simulink model "ADS_v1"  (R2026a)
settings: Solver=FixedStepDiscrete  StopTime=3600  FixedStep=ADS_P.dt
PostLoadFcn:
  | run(fullfile(fileparts(get_param('ADS_v1', 'FileName')), 'ads_setup.m'));
InitFcn:
  | run(fullfile(fileparts(get_param('ADS_v1', 'FileName')), 'ads_setup.m'));
values from neighbouring files (symbols this model uses):
  ADS_P = ads_params()    [ads_setup.m]
settings Model: Creator=Administrator  LastModifiedBy=Administrator

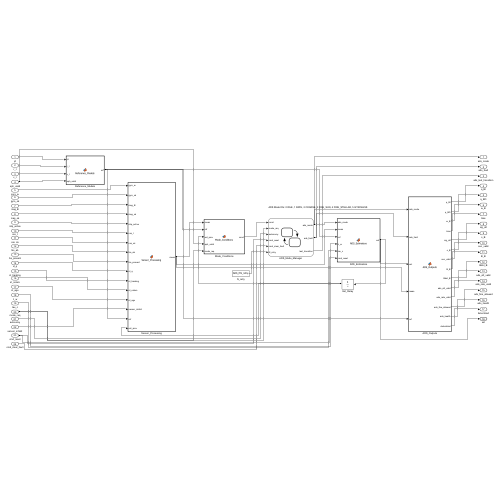
[thumbnail: Simulink's stored preview of the top-level diagram]
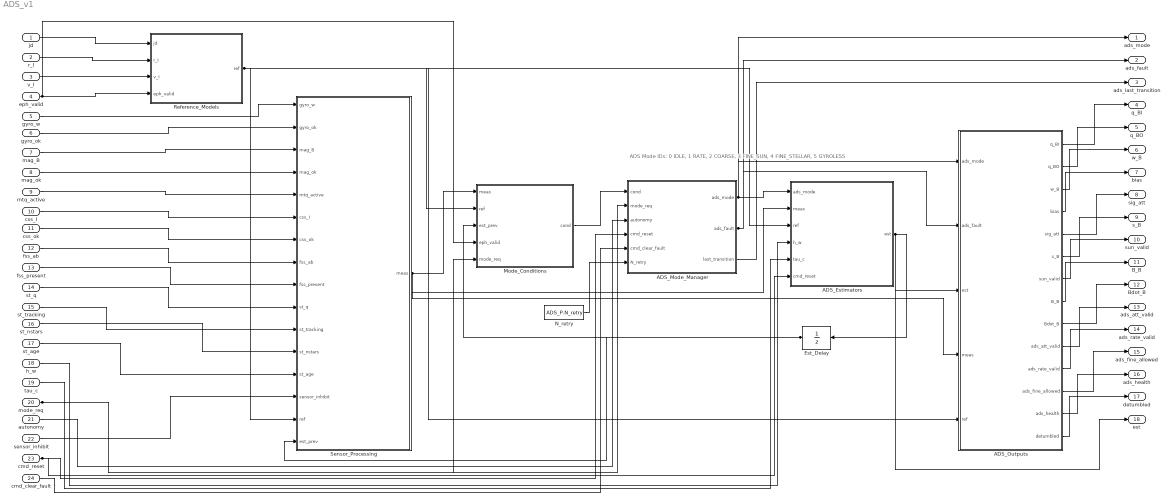
== system ADS_v1 ==
  note: ADS Mode IDs: 0 IDLE, 1 RATE, 2 COARSE, 3 FINE_SUN, 4 FINE_STELLAR, 5 GYROLESS
  jd : Inport  OutDataTypeStr=double  PortDimensions=1
  r_I : Inport  Port=2  OutDataTypeStr=double  PortDimensions=3
  v_I : Inport  Port=3  OutDataTypeStr=double  PortDimensions=3
  eph_valid : Inport  Port=4  OutDataTypeStr=boolean  PortDimensions=1
  gyro_w : Inport  Port=5  OutDataTypeStr=double  PortDimensions=3
  gyro_ok : Inport  Port=6  OutDataTypeStr=boolean  PortDimensions=1
  mag_B : Inport  Port=7  OutDataTypeStr=double  PortDimensions=3
  mag_ok : Inport  Port=8  OutDataTypeStr=boolean  PortDimensions=1
  mtq_active : Inport  Port=9  OutDataTypeStr=boolean  PortDimensions=1
  css_I : Inport  Port=10  OutDataTypeStr=double  PortDimensions=6
  css_ok : Inport  Port=11  OutDataTypeStr=boolean  PortDimensions=1
  fss_ab : Inport  Port=12  OutDataTypeStr=double  PortDimensions=4
  fss_present : Inport  Port=13  OutDataTypeStr=boolean  PortDimensions=2
  st_q : Inport  Port=14  OutDataTypeStr=double  PortDimensions=4
  st_tracking : Inport  Port=15  OutDataTypeStr=boolean  PortDimensions=1
  st_nstars : Inport  Port=16  OutDataTypeStr=double  PortDimensions=1
  st_age : Inport  Port=17  OutDataTypeStr=double  PortDimensions=1
  h_w : Inport  Port=18  OutDataTypeStr=double  PortDimensions=3
  tau_c : Inport  Port=19  OutDataTypeStr=double  PortDimensions=3
  mode_req : Inport  Port=20  OutDataTypeStr=uint8  PortDimensions=1
  autonomy : Inport  Port=21  OutDataTypeStr=boolean  PortDimensions=1
  sensor_inhibit : Inport  Port=22  OutDataTypeStr=uint8  PortDimensions=1
  cmd_reset : Inport  Port=23  OutDataTypeStr=boolean  PortDimensions=1
  cmd_clear_fault : Inport  Port=24  OutDataTypeStr=boolean  PortDimensions=1
  ADS_Estimators : MATLAB Function  TreatAsAtomicUnit=on
  ADS_Mode_Manager : Stateflow chart  TreatAsAtomicUnit=on
  ADS_Outputs : MATLAB Function  TreatAsAtomicUnit=on
  Est_Delay : UnitDelay  SampleTime=-1
  Mode_Conditions : MATLAB Function  TreatAsAtomicUnit=on
  N_retry : Constant  Value=ADS_P.N_retry  OutDataTypeStr=double  SampleTime=-1
  Reference_Models : MATLAB Function  TreatAsAtomicUnit=on
  Sensor_Processing : MATLAB Function  TreatAsAtomicUnit=on
  ads_mode : Outport
  ads_fault : Outport  Port=2
  ads_last_transition : Outport  Port=3
  q_BI : Outport  Port=4
  q_BO : Outport  Port=5
  w_B : Outport  Port=6
  bias : Outport  Port=7
  sig_att : Outport  Port=8
  s_B : Outport  Port=9
  sun_valid : Outport  Port=10
  B_B : Outport  Port=11
  Bdot_B : Outport  Port=12
  ads_att_valid : Outport  Port=13
  ads_rate_valid : Outport  Port=14
  ads_fine_allowed : Outport  Port=15
  ads_health : Outport  Port=16
  detumbled : Outport  Port=17
  est : Outport  Port=18  OutDataTypeStr=Bus: ADS_EstBus
  wires:
  jd/1 -> Reference_Models/1(jd)
  r_I/1 -> Reference_Models/2(r_I)
  v_I/1 -> Reference_Models/3(v_I)
  eph_valid/1 -> Reference_Models/4(eph_valid), Mode_Conditions/4(eph_valid)
  gyro_w/1 -> Sensor_Processing/1(gyro_w)
  gyro_ok/1 -> Sensor_Processing/2(gyro_ok)
  mag_B/1 -> Sensor_Processing/3(mag_B)
  mag_ok/1 -> Sensor_Processing/4(mag_ok)
  mtq_active/1 -> Sensor_Processing/5(mtq_active)
  css_I/1 -> Sensor_Processing/6(css_I)
  css_ok/1 -> Sensor_Processing/7(css_ok)
  fss_ab/1 -> Sensor_Processing/8(fss_ab)
  fss_present/1 -> Sensor_Processing/9(fss_present)
  st_q/1 -> Sensor_Processing/10(st_q)
  st_tracking/1 -> Sensor_Processing/11(st_tracking)
  st_nstars/1 -> Sensor_Processing/12(st_nstars)
  st_age/1 -> Sensor_Processing/13(st_age)
  sensor_inhibit/1 -> Sensor_Processing/14(sensor_inhibit)
  Reference_Models/1(ref) -> Sensor_Processing/15(ref), Mode_Conditions/2(ref), ADS_Estimators/3(ref), ADS_Outputs/5(ref)
  Est_Delay/1 -> Sensor_Processing/16(est_prev), Mode_Conditions/3(est_prev)
  Sensor_Processing/1(meas) -> Mode_Conditions/1(meas), ADS_Estimators/2(meas), ADS_Outputs/4(meas)
  mode_req/1 -> Mode_Conditions/5(mode_req), ADS_Mode_Manager/2(mode_req)
  Mode_Conditions/1(cond) -> ADS_Mode_Manager/1(cond)
  autonomy/1 -> ADS_Mode_Manager/3(autonomy)
  cmd_reset/1 -> ADS_Mode_Manager/4(cmd_reset), ADS_Estimators/6(cmd_reset)
  cmd_clear_fault/1 -> ADS_Mode_Manager/5(cmd_clear_fault)
  N_retry/1 -> ADS_Mode_Manager/6(N_retry)
  ADS_Mode_Manager/1(ads_mode) -> ADS_Estimators/1(ads_mode), ADS_Outputs/1(ads_mode), ads_mode/1
  h_w/1 -> ADS_Estimators/4(h_w)
  tau_c/1 -> ADS_Estimators/5(tau_c)
  ADS_Estimators/1(est) -> Est_Delay/1, ADS_Outputs/3(est), est/1
  ADS_Mode_Manager/2(ads_fault) -> ADS_Outputs/2(ads_fault), ads_fault/1
  ADS_Mode_Manager/3(last_transition) -> ads_last_transition/1
  ADS_Outputs/1(q_BI) -> q_BI/1
  ADS_Outputs/2(q_BO) -> q_BO/1
  ADS_Outputs/3(w_B) -> w_B/1
  ADS_Outputs/4(bias) -> bias/1
  ADS_Outputs/5(sig_att) -> sig_att/1
  ADS_Outputs/6(s_B) -> s_B/1
  ADS_Outputs/7(sun_valid) -> sun_valid/1
  ADS_Outputs/8(B_B) -> B_B/1
  ADS_Outputs/9(Bdot_B) -> Bdot_B/1
  ADS_Outputs/10(ads_att_valid) -> ads_att_valid/1
  ADS_Outputs/11(ads_rate_valid) -> ads_rate_valid/1
  ADS_Outputs/12(ads_fine_allowed) -> ads_fine_allowed/1
  ADS_Outputs/13(ads_health) -> ads_health/1
  ADS_Outputs/14(detumbled) -> detumbled/1

== matlab function ADS_v1/Sensor_Processing ==
  data: gyro_w input; meas output Bus: ADS_MeasBus; gyro_ok input; mag_B input; mag_ok input; mtq_active input; css_I input; css_ok input; fss_ab input; fss_present input; st_q input; st_tracking input; st_nstars input; st_age input; sensor_inhibit input; ref input Bus: ADS_RefBus; est_prev input Bus: ADS_EstBus; ADS_P parameter
function meas = Sensor_Processing(gyro_w, gyro_ok, mag_B, mag_ok, mtq_active, css_I, css_ok, fss_ab, fss_present, st_q, st_tracking, st_nstars, st_age, sensor_inhibit, ref, est_prev, ADS_P)
% Calibration, frame transformation and validity checks (Sections 3, 12.1).
meas = ads_sensor_processing(gyro_w, gyro_ok, mag_B, mag_ok, mtq_active, css_I, css_ok, fss_ab, fss_present, st_q, st_tracking, st_nstars, st_age, sensor_inhibit, ref, est_prev, ADS_P);

== matlab function ADS_v1/Reference_Models ==
  data: jd input; ref output Bus: ADS_RefBus; r_I input; v_I input; eph_valid input; ADS_P parameter
function ref = Reference_Models(jd, r_I, v_I, eph_valid, ADS_P)
% Sun, eclipse, IGRF field and LVLH frame (Section 3.7).
ref = ads_reference_models(jd, r_I, v_I, eph_valid, ADS_P);

== matlab function ADS_v1/Mode_Conditions ==
  data: meas input Bus: ADS_MeasBus; cond output Bus: ADS_CondBus; ref input Bus: ADS_RefBus; est_prev input Bus: ADS_EstBus; eph_valid input; mode_req input; ADS_P parameter
function cond = Mode_Conditions(meas, ref, est_prev, eph_valid, mode_req, ADS_P)
% Persistence-filtered guard conditions for transitions T1-T15 (Section 4.3).
cond = ads_mode_conditions(meas, ref, est_prev, eph_valid, mode_req, ADS_P);

== stateflow chart ADS_v1/ADS_Mode_Manager ==
  settings: enableNonTerminalStates=1
  state ADS_ACTIVE
    state ADS_FINE_STELLAR
      entry: ads_mode = uint8(4);
      during: bookkeeping();
    state ADS_FINE_SUN
      entry: ads_mode = uint8(3);
      during: bookkeeping();
    state ADS_COARSE
      entry: ads_mode = uint8(2);
      during: bookkeeping();
    state ADS_GYROLESS
      entry: ads_mode = uint8(5);
      during: bookkeeping();
    state ADS_RATE
      entry: ads_mode = uint8(1);
      during: bookkeeping();
    ADS_FINE_STELLAR -> ADS_GYROLESS [order 1] : [T11()]{fault_fb(11)}
    ADS_COARSE -> ADS_FINE_STELLAR [order 5] : [T10()]{mark(10)}
    (junction 73) -> ADS_FINE_STELLAR [order 1] : [T14_FST()]{mark(14)}
    ADS_RATE -> ADS_FINE_STELLAR [order 1] : [T10()]{mark(10)}
    ADS_FINE_STELLAR -> ADS_COARSE [order 2] : [T9f()]{fault_fb(9)}
    ADS_FINE_STELLAR -> ADS_COARSE [order 4] : [T9g()]{mark(9)}
    ADS_FINE_SUN -> ADS_FINE_STELLAR [order 5] : [T7()]{mark(7)}
    ADS_FINE_STELLAR -> (junction 72) [order 5] : [cond.req_rank < 5]{mark(16)}
    ADS_FINE_STELLAR -> ADS_FINE_SUN [order 3] : [T8()]{mark(8)}
    (junction 73) -> ADS_FINE_SUN [order 2] : [T14_FSUN()]{mark(14)}
    (junction 73) -> ADS_COARSE [order 3] : [T14_CRS()]{mark(14)}
    ADS_GYROLESS -> (junction 73) [order 4] : [T14()]
    ADS_FINE_SUN -> ADS_GYROLESS [order 1] : [T11()]{fault_fb(11)}
    (default) -> ADS_RATE
    ADS_COARSE -> ADS_FINE_SUN [order 6] : [T5()]{mark(5)}
    ADS_FINE_SUN -> ADS_COARSE [order 3] : [T6g()]{mark(6)}
    ADS_FINE_SUN -> (junction 72) [order 4] : [cond.req_rank < 4]{mark(16)}
    ADS_FINE_SUN -> ADS_COARSE [order 2] : [T6f()]{fault_fb(6)}
    (junction 72) -> ADS_FINE_SUN [order 4] : [mode_req == uint8(3)]
    ADS_COARSE -> ADS_GYROLESS [order 1] : [T11()]{fault_fb(11)}
    (junction 72) -> ADS_COARSE [order 3] : [mode_req == uint8(2)]
    (junction 72) -> ADS_GYROLESS [order 2] : [mode_req == uint8(5)]
    ADS_COARSE -> (junction 72) [order 4] : [cond.req_rank < 3]{mark(16)}
    ADS_RATE -> ADS_COARSE [order 2] : [T3()]{mark(3)}
    ADS_COARSE -> ADS_RATE [order 3] : [T4g()]{mark(4)}
    ADS_COARSE -> ADS_RATE [order 2] : [T4f()]{fault_fb(4)}
    ADS_RATE -> ADS_GYROLESS [order 3] : [T12()]{mark(12)}
    ADS_GYROLESS -> ADS_RATE [order 1] : [T13f()]{fault_fb(13)}
    ADS_GYROLESS -> ADS_RATE [order 2] : [T13g()]{mark(13)}
    ADS_GYROLESS -> (junction 72) [order 3] : [cond.req_rank < 2]{mark(16)}
    (junction 72) -> ADS_RATE [order 1] : [mode_req == uint8(1)]
  note: ADS mode manager (ADCS-ADS-DD-001, Section 4)
      | Mode IDs: 0 IDLE, 1 RATE, 2 COARSE, 3 FINE_SUN, 4 FINE_STELLAR, 5 GYROLESS
      | Guard functions T1..T15 = document Table 6 (f = fault-driven, g = geometric).
      | Execution order: T15 > gyro failure > fault > geometric > downgrade > upgrade.
      | Super-step semantics give the same-cycle fallback cascade.
      | last_transition = document transition ID, 16 = commanded downgrade.
  state ADS_IDLE
    entry: ads_mode = uint8(0);
    during: bookkeeping();
  (default) -> ADS_IDLE
  ADS_RATE -> ADS_IDLE [order 4] : [T2()]{fault_fb(2)}
  ADS_IDLE -> ADS_RATE : [T1()]{mark(1)}
  ADS_ACTIVE -> ADS_IDLE : [T15()]{mark(15)}
  data: id function_input double; id function_input double; y function_output boolean; y function_output boolean; y function_output boolean; y function_output boolean; y function_output boolean; y function_output boolean; y function_output boolean; y function_output boolean; y function_output boolean; y function_output boolean; y function_output boolean; y function_output boolean; y function_output boolean; y function_output boolean; y function_output boolean; y function_output boolean; y function_output boolean; y function_output boolean; y function_output boolean; y function_output boolean; y function_output boolean; y function_output boolean; y function_output boolean; cond input Bus: ADS_CondBus; mode_req input uint8; autonomy input boolean; cmd_reset input boolean; cmd_clear_fault input boolean; N_retry input double; ads_mode output uint8 =0; ads_fault output boolean =0; last_transition output uint8 =0; retry_cnt local double =0; clear_cnt local double =0
  function bookkeeping:
    | function bookkeeping()
    | % Retry timer and ads_fault latch (Sections 4.4, 12.4); runs every cycle.
    | retry_cnt = max(retry_cnt - 1, 0);
    | if cmd_clear_fault
    |     ads_fault = false;  clear_cnt = 0;
    | elseif ads_fault && ads_mode == mode_req && retry_cnt == 0
    |     clear_cnt = clear_cnt + 1;
    |     if clear_cnt >= N_retry
    |         ads_fault = false;  clear_cnt = 0;
    |     end
    | else
    |     clear_cnt = 0;
    | end
    | end
  function mark(id):
    | function mark(id)
    | % Record the document transition ID (16 = commanded downgrade).
    | last_transition = uint8(id);
    | if id == 15 && cond.num_fault
    |     ads_fault = true;
    | end
    | end
  function fault_fb(id):
    | function fault_fb(id)
    | % Fault-driven fallback: latch ads_fault and inhibit upgrades for N_retry cycles.
    | last_transition = uint8(id);
    | ads_fault = true;
    | retry_cnt = N_retry;
    | end
  function y = up:
    | function y = up()
    | % Upgrades allowed: autonomy enabled and retry timer expired (document Table 6)
    | y = autonomy && retry_cnt == 0;
    | end
  function y = T1:
    | function y = T1()
    | % IDLE -> RATE (document Table 6)
    | y = ~cmd_reset && autonomy && mode_req ~= uint8(0) && (cond.gyr_ok || cond.mag_ok);
    | end
  function y = T2:
    | function y = T2()
    | % RATE -> IDLE (fault) (document Table 6)
    | y = cond.rate_src_lost;
    | end
  function y = T3:
    | function y = T3()
    | % RATE -> COARSE (document Table 6)
    | y = up() && cond.req_rank >= 3 && cond.gyr_ok && cond.mag_ok && cond.eph_ok && cond.w_lt_C_in && cond.triad_ok;
    | end
  function y = T4f:
    | function y = T4f()
    | % COARSE -> RATE (fault) (document Table 6)
    | y = cond.gyr_lost || cond.mag_lost || cond.eph_lost || cond.coarse_fault;
    | end
  function y = T4g:
    | function y = T4g()
    | % COARSE -> RATE (rate too high) (document Table 6)
    | y = cond.w_gt_C_out;
    | end
  function y = T5:
    | function y = T5()
    | % COARSE -> FINE_SUN (document Table 6)
    | y = up() && cond.req_rank >= 4 && cond.coarse_conv && cond.sig_lt_FS_in && cond.fss_ok && cond.mag_ok && cond.w_lt_FS_in;
    | end
  function y = T6f:
    | function y = T6f()
    | % FINE_SUN -> COARSE (fault) (document Table 6)
    | y = cond.gyr_lost || cond.mag_lost || cond.eph_lost || cond.fine_sun_fault;
    | end
  function y = T6g:
    | function y = T6g()
    | % FINE_SUN -> COARSE (no FSS / rate) (document Table 6)
    | y = cond.fss_lost || cond.w_gt_FS_out;
    | end
  function y = T7:
    | function y = T7()
    | % FINE_SUN -> FINE_STELLAR (document Table 6)
    | y = up() && cond.req_rank >= 5 && cond.st_ok && cond.w_lt_ST_in && ~cond.st_suspect;
    | end
  function y = T8:
    | function y = T8()
    | % FINE_STELLAR -> FINE_SUN (document Table 6)
    | y = (cond.st_lost || cond.w_gt_ST_out || cond.st_suspect) && cond.fss_ok && cond.mag_ok && cond.eph_ok;
    | end
  function y = T9f:
    | function y = T9f()
    | % FINE_STELLAR -> COARSE (fault) (document Table 6)
    | y = cond.gyr_lost || cond.stellar_fault;
    | end
  function y = T9g:
    | function y = T9g()
    | % FINE_STELLAR -> COARSE (ST out) (document Table 6)
    | y = cond.st_lost || cond.w_gt_ST_out || cond.st_suspect;
    | end
  function y = T10:
    | function y = T10()
    | % RATE/COARSE -> FINE_STELLAR (document Table 6)
    | y = up() && cond.req_rank >= 5 && cond.gyr_ok && cond.st_ok && cond.w_lt_ST_in;
    | end
  function y = T11:
    | function y = T11()
    | % COARSE/FINE_SUN/FINE_STELLAR -> GYROLESS (document Table 6)
    | y = cond.gyr_lost && cond.gyroless_en && cond.gl_init_ok;
    | end
  function y = T12:
    | function y = T12()
    | % RATE -> GYROLESS (document Table 6)
    | y = up() && cond.req_rank >= 2 && cond.gyr_lost && cond.gyroless_en && cond.mag_ok && cond.w_lt_GL_in && cond.gl_init_ok;
    | end
  function y = T13f:
    | function y = T13f()
    | % GYROLESS -> RATE (fault) (document Table 6)
    | y = cond.gl_meas_lost || cond.gl_fault;
    | end
  function y = T13g:
    | function y = T13g()
    | % GYROLESS -> RATE (rate too high) (document Table 6)
    | y = cond.w_gt_GL_out;
    | end
  function y = T14:
    | function y = T14()
    | % GYROLESS -> gyro modes (gyro recovered) (document Table 6)
    | y = cond.gyr_recovered && cond.req_rank >= 3;
    | end
  function y = T14_FST:
    | function y = T14_FST()
    | % T14 target FINE_STELLAR (document Table 6)
    | y = cond.req_rank >= 5 && cond.st_ok && cond.w_lt_ST_in;
    | end
  function y = T14_FSUN:
    | function y = T14_FSUN()
    | % T14 target FINE_SUN (document Table 6)
    | y = cond.req_rank >= 4 && cond.fss_ok && cond.mag_ok && cond.eph_ok && cond.sig_lt_FS_in && cond.w_lt_FS_in;
    | end
  function y = T14_CRS:
    | function y = T14_CRS()
    | % T14 target COARSE (document Table 6)
    | y = cond.mag_ok && cond.eph_ok;
    | end
  function y = T15:
    | function y = T15()
    | % Any -> IDLE (command / numerical fault) (document Table 6)
    | y = cmd_reset || mode_req == uint8(0) || cond.num_fault;
    | end

== matlab function ADS_v1/ADS_Estimators ==
  data: ads_mode input; est output Bus: ADS_EstBus; meas input Bus: ADS_MeasBus; ref input Bus: ADS_RefBus; h_w input; tau_c input; cmd_reset input; ADS_P parameter
function est = ADS_Estimators(ads_mode, meas, ref, h_w, tau_c, cmd_reset, ADS_P)
% Estimator of the active mode with hand-over rules (Sections 5-11, Table 8).
est = ads_estimator(ads_mode, meas, ref, h_w, tau_c, cmd_reset, ADS_P);

== matlab function ADS_v1/ADS_Outputs ==
  data: ads_mode input; q_BI output; ads_fault input; est input Bus: ADS_EstBus; meas input Bus: ADS_MeasBus; ref input Bus: ADS_RefBus; q_BO output; w_B output; bias output; sig_att output; s_B output; sun_valid output; B_B output; Bdot_B output; ads_att_valid output; ads_rate_valid output; ads_fine_allowed output; ads_health output; detumbled output; ADS_P parameter
function [q_BI, q_BO, w_B, bias, sig_att, s_B, sun_valid, B_B, Bdot_B, ads_att_valid, ads_rate_valid, ads_fine_allowed, ads_health, detumbled] = ADS_Outputs(ads_mode, ads_fault, est, meas, ref, ADS_P)
% ADS outputs and status flags (Table 9).
[q_BI, q_BO, w_B, bias, sig_att, s_B, sun_valid, B_B, Bdot_B, ads_att_valid, ads_rate_valid, ads_fine_allowed, ads_health, detumbled] = ads_outputs(ads_mode, ads_fault, est, meas, ref, ADS_P);
